simulink model "TP2_commande_des_clignotants_Simulink"  (R2022b)
settings: Solver=VariableStepAuto  StartTime=0.0  StopTime=10.0  RelTol=1e-3
libraries: simulink x8
settings Model: Creator=HP  LastModifiedBy=HP

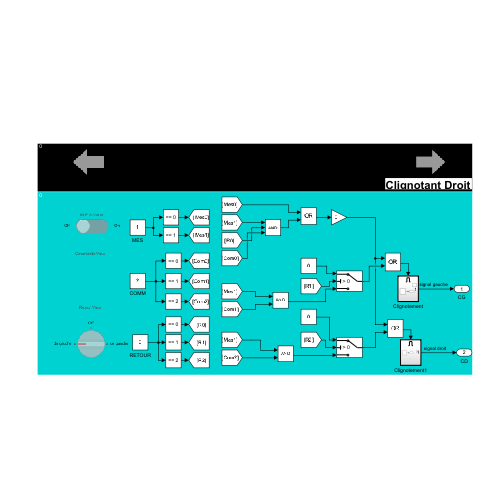
[thumbnail: Simulink's stored preview of the top-level diagram]
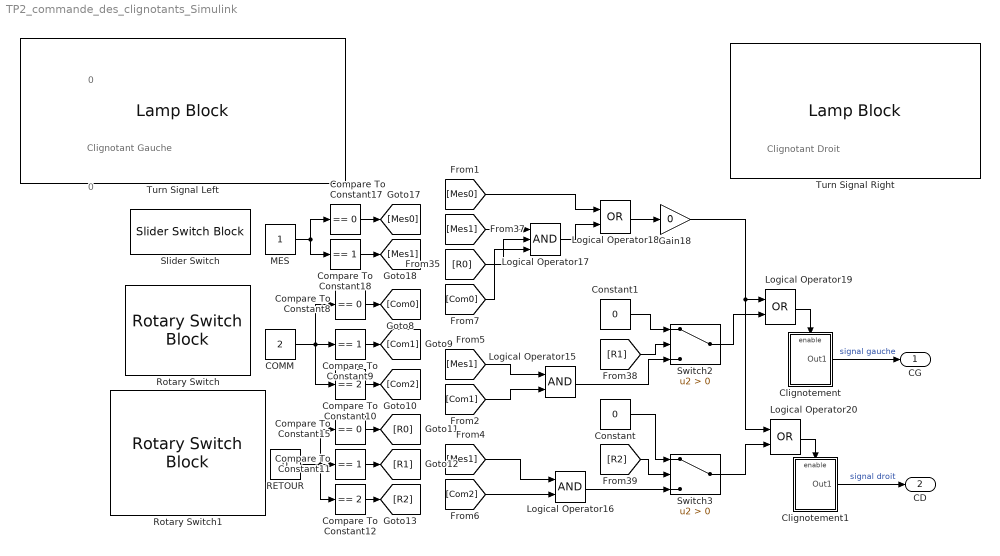
== system TP2_commande_des_clignotants_Simulink ==
  note: Clignotant Droit
  note: 0
  note: 0
  note: Clignotant Gauche
  COMM : Constant  Value=2
  Clignotement : Subsystem
  Clignotement1 : Subsystem
  Compare To Constant10 : simulink/Logic and Bit Operations/Compare To Constant  relop===  const=2  OutDataTypeStr=boolean
  Compare To Constant11 : simulink/Logic and Bit Operations/Compare To Constant  relop===  const=1  OutDataTypeStr=boolean
  Compare To Constant12 : simulink/Logic and Bit Operations/Compare To Constant  relop===  const=2  OutDataTypeStr=boolean
  Compare To Constant15 : simulink/Logic and Bit Operations/Compare To Constant  relop===  const=0  OutDataTypeStr=boolean
  Compare To Constant17 : simulink/Logic and Bit Operations/Compare To Constant  relop===  const=0  OutDataTypeStr=boolean
  Compare To Constant18 : simulink/Logic and Bit Operations/Compare To Constant  relop===  const=1  OutDataTypeStr=boolean
  Compare To Constant8 : simulink/Logic and Bit Operations/Compare To Constant  relop===  const=0  OutDataTypeStr=boolean
  Compare To Constant9 : simulink/Logic and Bit Operations/Compare To Constant  relop===  const=1  OutDataTypeStr=boolean
  Constant : Constant  Value=0
  Constant1 : Constant  Value=0
  Gain18 : Gain  Gain=0
  Logical Operator15 : Logic  AllPortsSameDT=off  OutDataTypeStr=boolean
  Logical Operator16 : Logic  AllPortsSameDT=off  OutDataTypeStr=boolean
  Logical Operator17 : Logic  Inputs=3  AllPortsSameDT=off  OutDataTypeStr=boolean
  Logical Operator18 : Logic  Operator=OR  AllPortsSameDT=off  OutDataTypeStr=boolean
  Logical Operator19 : Logic  Operator=OR  AllPortsSameDT=off  OutDataTypeStr=boolean
  Logical Operator20 : Logic  Operator=OR  AllPortsSameDT=off  OutDataTypeStr=boolean
  MES : Constant
  RETOUR : Constant  Value=0
  Rotary Switch : RotarySwitchBlock
      settings: Values={{'Gauche', 'Off', 'Droite'}, [1 0 2]}
  Rotary Switch1 : RotarySwitchBlock
      settings: Values={{'de gauche', 'Off', 'de gauche'}, [1 0 2]}
  Slider Switch : SliderSwitchBlock
      settings: Values={{'Off', 'On'}, [0 1]}
  Switch2 : Switch  Criteria=u2 > Threshold  SaturateOnIntegerOverflow=off  InputSameDT=off
  Switch3 : Switch  Criteria=u2 > Threshold  SaturateOnIntegerOverflow=off  InputSameDT=off
  Turn Signal Left : LampBlock  LabelPosition=Hide  Icon=TurnSignalLeft
  Turn Signal Right : LampBlock  LabelPosition=Hide  Icon=TurnSignalRight
  CG : Outport
  CD : Outport  Port=2
  wires:
  Logical Operator16/1 -> Switch3/3
  [Mes0] -> Logical Operator18/1
  Constant/1 -> Switch3/1
  [Mes1] -> Logical Operator16/1
  Compare To Constant18/1 -> [Mes1]
  Compare To Constant9/1 -> [Com1]
  Compare To Constant15/1 -> [R0]
  [Com2] -> Logical Operator16/2
  Logical Operator17/1 -> Logical Operator18/2
  [Com0] -> Logical Operator17/3
  [R0] -> Logical Operator17/2
  Compare To Constant17/1 -> [Mes0]
  [Com1] -> Logical Operator15/2
  RETOUR/1 -> Compare To Constant15/1, Compare To Constant12/1, Compare To Constant11/1
  Compare To Constant12/1 -> [R2]
  [R1] -> Switch2/2
  Compare To Constant8/1 -> [Com0]
  [Mes1] -> Logical Operator17/1
  Compare To Constant10/1 -> [Com2]
  COMM/1 -> Compare To Constant8/1, Compare To Constant9/1, Compare To Constant10/1
  Constant1/1 -> Switch2/1
  [R2] -> Switch3/2
  Clignotement1/1(Out1) -> CD/1  "signal droit"
  Switch3/1 -> Logical Operator20/2
  Gain18/1 -> Logical Operator19/1, Logical Operator20/1
  [Mes1] -> Logical Operator15/1
  MES/1 -> Compare To Constant17/1, Compare To Constant18/1
  Logical Operator15/1 -> Switch2/3
  Switch2/1 -> Logical Operator19/2
  Clignotement/1(Out1) -> CG/1  "signal gauche"
  Compare To Constant11/1 -> [R1]
  Logical Operator20/1 -> Clignotement1/Enable
  Logical Operator19/1 -> Clignotement/Enable
  Logical Operator18/1 -> Gain18/1

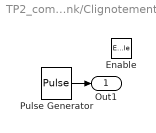
== system TP2_commande_des_clignotants_Simulink/Clignotement ==
  Enable : EnablePort
  Pulse Generator : DiscretePulseGenerator  PulseType=Time based  PulseWidth=50
  Out1 : Outport
  wires:
  Pulse Generator/1 -> Out1/1

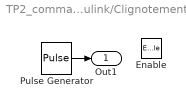
== system TP2_commande_des_clignotants_Simulink/Clignotement1 ==
  Enable : EnablePort
  Pulse Generator : DiscretePulseGenerator  PulseType=Time based  PulseWidth=50
  Out1 : Outport
  wires:
  Pulse Generator/1 -> Out1/1
